simulink model "PMSM_SMO_ClosedLoop"  (R2026a)
settings: Solver=ode4  StopTime=.5  FixedStep=timing_h  MaxStep=1e-6
InitFcn:
  | pmsm_sensorless_v2_init(bdroot);
model workspace (MATLAB code in the model file + MAT data in the model file):
  T = 1e-6    (= 1e-06)
  MotorProfile = 'CHENSHA 200W / firmware profile revision 2'
  MotorSourceCommit = '48d6e86814ac6657b1313b4c92ef24c88f492e07'
  Pn = 200
  Un = 24
  Vdc = 24
  I_rated_rms = 11.5
  I_peak_rms = 23
  In = sqrt(2)*I_rated_rms
  I_peak = sqrt(2)*I_peak_rms
  n = 3000
  p = 5
  Rs = 0.105125
  Ld = 103.7615e-6    (= 0.0001037615)
  Lq = 103.7615e-6    (= 0.0001037615)
  Ls = Ld    (= 0.0001037615)
  phis = 0.06/(sqrt(2)*1.5*p)
  J = 32e-6    (= 3.2e-05)
  F = 0
  Kt = 1.5*p*phis
  Tn = 0.69
  T_peak = 1.38
  Iq_limit = 8
  accel_limit_rad_s2 = 1200
  speed_peak_rad_s = 335
  I_protection_A = 10
  Vbus_protection_high_V = 30
  Vbus_protection_low_V = 10
  RE = 10000
  rr = 2*pi/RE    (= 0.000628318530718)
  encoder_direction = -1
  fN = p*n/60    (= 250)
  wN = 2*pi*fN    (= 1570.79632679)
  ki_p = 0.8
  ki_i = 1
  fc = 20e3    (= 20000)
  Ts = 1/fc    (= 5e-05)
  dt = Ts    (= 5e-05)
  Ts_speed = 2*dt    (= 0.0001)
  w_sb = 2*pi*fN*1.2    (= 1884.95559215)
  fcb = 1000
  fwb = 50
  wc = 2*pi*fcb    (= 6283.18530718)
  wsc = 2*pi*fwb    (= 314.159265359)
  K = 30/pi    (= 9.54929658551)
  kp_w = 0.00069087230807625508    (= 0.000690872308076)
  ki_w = 0.04340878735241975    (= 0.0434087873524)
  ks_w = 0.98718608264211138    (= 0.987186082642)
  kp_id = 0.7539822368615503    (= 0.753982236862)
  ki_id = 879.64594300514204    (= 879.645943005)
  ks_id = 1.1309733552923253    (= 1.13097335529)
  kp_iq = 0.7539822368615503    (= 0.753982236862)
  ki_iq = 879.64594300514204    (= 879.645943005)
  ks_iq = 1.1309733552923253    (= 1.13097335529)
  Bm = 0
  uplimit_w = Kt*Iq_limit
  downlimit_w = -uplimit_w
  uplimit_id = Vdc/sqrt(3)
  downlimit_id = -uplimit_id
  uplimit_iq = Vdc/sqrt(3)
  downlimit_iq = -uplimit_iq
  teaching_Ts_speed = Ts_speed    (= 0.0001)
  teach_pwm_on = 0
  teach_pwm_cycles = 1
  decoupling_enabled = 1
  voltage_utilization = 0.96
  timing_on = 0
  timing_h = 1e-6    (= 1e-06)
  timing_control_sample = dt    (= 5e-05)
  timing_speed_sample = Ts_speed    (= 0.0001)
  timing_static_math = -1
  timing_carrier_y = [0 Ts/2 0]
  timing_adc_cfg = [0 0 0 1e-6 Ts 24.375e-6 1.1875e-6 1.5e-6 0 .5e-6 2]
  timing_pwm_cfg = [0 1e-6 Ts 24.375e-6 1.1875e-6 1.5e-6 0 5e-6 0 4000]
  dead_gate_on = 0
  dead_h = 1e-6    (= 1e-06)
  dead_gate_cfg = [0 1e-6 .5e-6]
  dead_comp_cfg = [0 .5e-6 Ts .05]
  dead_bridge_cfg = [p phis .01 0 .01 .7]
  sless_adc_mode = [1 0]
  sless_cfg = [0.105125 0.0001037615 5e-05 0.950604638176 0.469872645179 70 14 0.2 0.028048810878 0.777767679172 1332.66360365 888264.396098 2000 5 2 1.5 0.5 0.15]
  sless_closed_cfg = [5e-05 2.8875e-05 5 0.04 0.06 0.14 1200 6 6 0.18 0.02 0.04 0.02 0.08 0.000690872308076 0.0434087873524 0.987186082642 0.33941125497 0.0424264068712 2]
  sless_direction = 1
  sless_enabled = 1
  sless_v2_cfg = [6.25e-08 5e-05 0.0001 2.4375e-05 1.1875e-06 1.5e-06 0 0 3e-06 5e-06 2e-06 6e-05 7.5e-05 4.375e-07 0.012 0.6 0.05 0.05 5 2000 0.105125 0.0001037615 4500 2000 1.008 0.994 1.002 0.04 -0.02 0.005 20 12 0 0 0.25]
  sless_v2_interference_s = 0
  sless_voltage_cfg = [6.25e-08 5e-05 2.8875e-05 0.105125 0.0001037615 1]
undefined symbols (not defined in the file): DiscIntNeverNeededParam
libraries: simulink x3
(part 1 of 3)
Description:
  | CHENSHA 200W nominal motor profile from AxDr_L dev 48d6e86814ac6657b1313b4c92ef24c88f492e07. PI gains frozen from previous model. Current/PWM 20kHz, speed 10kHz. Bench iq command limit 8A. ABZ estimator, active protection and hardware sampling windows are not implemented.
settings Model: Creator=OptiPlex 7090  LastModifiedBy=lenovo
settings SimscapeCC: SimscapeLogDecimation=1  SimscapeNominalValues="[{\"value\":\"1\",\"unit\":\"A\"},{\"value\":\"1\",\"unit\":\"bar\"},{\"value\":\"1\",\"unit\":\"cm^2\"},{\"value\":\"1\",\"unit\":\"cm^3/s\"},{\"value\":\"1\",\"unit\":\"kJ/kg\"},{\"value\":\"1\",\"unit\":\"kW\"},{\"value\":\"1\",\"unit\":\"l\"},{\"value\":\"1\",\"unit\":\"N\"},{\"value\":\"1\",\"unit\":\"N*m\"},{\"value\":\"1\",\"unit\":\"V\"}]"  SimscapeLogDataHistory=5000  SimscapeLogType=none

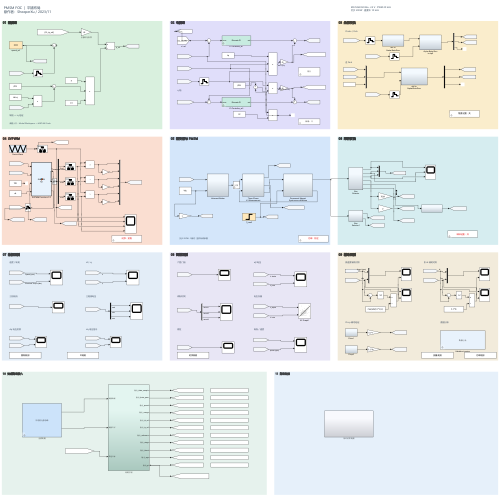
[thumbnail: Simulink's stored preview of the top-level diagram]
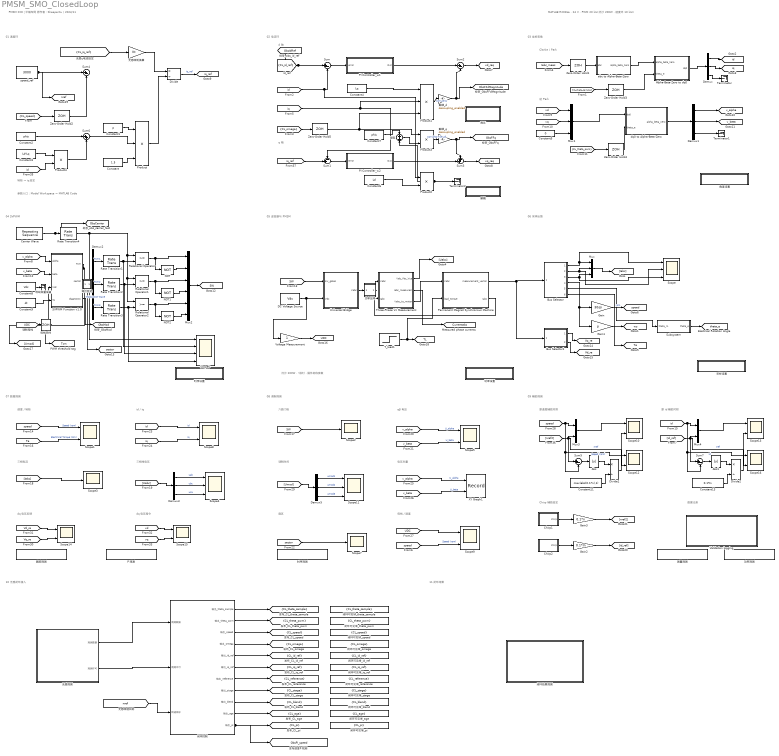
== system PMSM_SMO_ClosedLoop ==
  note: 参数入口：Model Workspace → MATLAB Code
  note: 07 数据观测
  note: 04 SVPWM
  note: 01 速度环
  note: 沉沙 200W · 5极对 · 固件标称参数
  note: 02 电流环
  note: 03 坐标变换
  note: 05 逆变器与 PMSM
  note: PMSM FOC  |  平铺布局
      | 原作者：SheeperXu / 2023/11
  note: 06 采样反馈
  note: MATLAB R2026a · 24 V · PWM 20 kHz
      | 沉沙 200W · 速度环 10 kHz
  note: 08 调制观测
  note: 09 辅助观测
  note: Clarke / Park
  note: 逆 Park
  note: d 轴
  note: q 轴
  note: 转矩 → iq 给定
  note: 速度 / 转矩
  note: id / iq
  note: 三相电流
  note: 三相线电压
  note: dq 电压反馈
  note: dq 电压指令
  note: 六路门极
  note: αβ 电压
  note: 调制时间
  note: 电压矢量
  note: 扇区
  note: 母线 / 速度
  note: 原速度辅助对照
  note: 原 id 辅助对照
  note: Chirp 辅助给定
  note: 数据记录
  note: 10 无感闭环接入
  note: 11 闭环结果
  Abs : Abs  SaturateOnIntegerOverflow=off
  Abs1 : Abs  SaturateOnIntegerOverflow=off
  Alpha-Beta-Zero to dq0 : Subsystem
  Bus Selector : Subsystem
  Bus Selector1 : Subsystem
  Carrier Wave : simulink/Sources/Repeating Sequence  rep_seq_t=[0 Ts/2 Ts]  rep_seq_y=timing_carrier_y
  Chirp1 : Subsystem
  Chirp2 : Subsystem
  Constant : Constant  Value=1.5
  Constant1 : Constant  Value=p
  Constant11 : Constant  Value=max(abs(0.1*n),1)
  Constant13 : Constant  Value=0.1*In
  Constant2 : Constant  Value=phis
  Constant3 : Constant  Value=Ld-Lq
  Constant4 : Constant  Value=Lq
  Constant5 : Constant  Value=0
  Constant6 : Constant  Value=Ld
  Constant7 : Constant  Value=phis
  Constant8 : Constant  Value=Vdc
  Constant9 : Constant  Value=dt
  DC Voltage Source : Constant  Value=Vdc
  Demux{,1..3,5} (5 alike) : Demux  Outputs=3
  Divide : Product  Inputs=*/
  Divide1 : Product  Inputs=*/
  Divide2 : Product  Inputs=*/
  Gain : Gain  Gain=30/pi
  Gain1 : Gain  Gain=p
  Gain2 : Gain  Gain=0.1*In
  Gain3 : Gain  Gain=0.1*n
  Mux : Mux  Inputs=3
  Mux1 : Mux  Inputs=3
  Mux2 : Mux  Inputs=6
  Mux3 : Mux  Inputs=2
  Mux4 : Mux  Inputs=2
  NOT : Logic  Operator=NOT  IconShape=distinctive  AllPortsSameDT=off  OutDataTypeStr=boolean
  NOT1 : Logic  Operator=NOT  IconShape=distinctive  AllPortsSameDT=off  OutDataTypeStr=boolean
  NOT2 : Logic  Operator=NOT  IconShape=distinctive  AllPortsSameDT=off  OutDataTypeStr=boolean
  PI Controller_w1 : Subsystem  mask{Kp=kp_id, Ki=ki_id, Ks=ks_id, uplimit=uplimit_id, downlimit=downlimit_id, SampleTime=timing_control_sample}
      mask prompts: uplimit "Up_Limit"; downlimit "Down_Limit"; SampleTime "Sample_Time(s)"
      mask DialogControl DescTextVar Prompt: PI Controller
      mask DialogControl ParameterGroupVar Prompt: 参数
      mask DialogControl Control2 Prompt: PI Controller Parameters
      mask Display:
      | disp('Discrete PI');
      | port_label('input',1,'error');
      | port_label('output',1,'out');
  PI Controller_w2 : Subsystem  mask{Kp=kp_iq, Ki=ki_iq, Ks=ks_iq, uplimit=uplimit_iq, downlimit=downlimit_iq, SampleTime=timing_control_sample}
      mask prompts: uplimit "Up_Limit"; downlimit "Down_Limit"; SampleTime "Sample_Time(s)"
      mask DialogControl DescTextVar Prompt: PI Controller
      mask DialogControl ParameterGroupVar Prompt: 参数
      mask DialogControl Control2 Prompt: PI Controller Parameters
      mask Display:
      | disp('Discrete PI');
      | port_label('input',1,'error');
      | port_label('output',1,'out');
  PI观测 : Subsystem  mask(PI观测){}
      mask help: 每组顺序：P / I / 限幅前 / 限幅后。速度环单位N*m；电流环单位V。
      settings: OpenFcn=open_system([gcb '/总览']);
      mask Display: disp('PI观测');
  Permanent Magnet Synchronous Machine : Subsystem
  Product : Product  Inputs=3  SampleTime=timing_static_math
  Product1 : Product  Inputs=3
  Product2 : Product
  Product3 : Product
  Product4 : Product
  Rate Transition{1..4} (4 alike) : RateTransition  Deterministic=off
  Relational Operator : RelationalOperator  OutDataTypeStr=boolean  RndMeth=Simplest  InputSameDT=off
  Relational Operator1 : RelationalOperator  OutDataTypeStr=boolean  RndMeth=Simplest  InputSameDT=off
  Relational Operator2 : RelationalOperator  OutDataTypeStr=boolean  RndMeth=Simplest  InputSameDT=off
  SVPWM Function v1.0 : MATLAB Function  TreatAsAtomicUnit=on
  Scope : Scope  NumInputPorts=3
      settings: ActiveDisplayYMinimum=-2.21804  ActiveDisplayYMaximum=2.01558
  Scope{1,5,8..10,12..16} (10 alike) : Scope  NumInputPorts=2
      Scope1 settings: ActiveDisplayYMinimum=-389.77916  ActiveDisplayYMaximum=3379.29942  DataLoggingVariableName=ScopeData3
      Scope10 settings: ActiveDisplayYMinimum=-396.87  ActiveDisplayYMaximum=406.58362  DataLoggingVariableName=ScopeData14
      Scope12 settings: ActiveDisplayYMinimum=-396.37475  ActiveDisplayYMaximum=405.982  DataLoggingVariableName=ScopeData15
      Scope13 settings: ActiveDisplayYMinimum=-1.103599846952628  ActiveDisplayYMaximum=7.8207274341227286  DataLoggingVariableName=ScopeData18
      Scope14 settings: ActiveDisplayYMinimum=-20.0031  ActiveDisplayYMaximum=19.99997  DataLoggingVariableName=ScopeData16
      Scope15 settings: ActiveDisplayYMinimum=-4.01522  ActiveDisplayYMaximum=14.86532  DataLoggingVariableName=ScopeData17
      Scope16 settings: ActiveDisplayYMinimum=-1.103599846952628  ActiveDisplayYMaximum=7.8207274341227286  DataLoggingVariableName=ScopeData19
      Scope5 settings: ActiveDisplayYMinimum=-10.001349433509255  ActiveDisplayYMaximum=9.60909342723076  DataLoggingVariableName=ScopeData7
      Scope8 settings: ActiveDisplayYMinimum=-0.61064  ActiveDisplayYMaximum=0.4372  DataLoggingVariableName=ScopeData10
      Scope9 settings: ActiveDisplayYMinimum=14  ActiveDisplayYMaximum=34  DataLoggingVariableName=ScopeData11
  Scope11 : Scope  NumInputPorts=3
      settings: ActiveDisplayYMinimum=2E-6  ActiveDisplayYMaximum=2.5E-5  DataLoggingVariableName=ScopeData13
  Scope2 : Scope
      settings: ActiveDisplayYMinimum=-0.125  ActiveDisplayYMaximum=1.125  DataLoggingVariableName=ScopeData4
  Scope3 : Scope
      settings: ActiveDisplayYMinimum=-14.55664  ActiveDisplayYMaximum=14.56696  DataLoggingVariableName=ScopeData5
  Scope4 : Scope  NumInputPorts=3
      settings: ActiveDisplayYMinimum=-30.00473  ActiveDisplayYMaximum=30.00442  DataLoggingVariableName=ScopeData6
  Scope6 : Scope  NumInputPorts=4
      settings: ActiveDisplayYMinimum=-3E-6  ActiveDisplayYMaximum=2.8E-5  DataLoggingVariableName=ScopeData8
  Scope7 : Scope
      settings: ActiveDisplayYMinimum=0.375  ActiveDisplayYMaximum=6.625  DataLoggingVariableName=ScopeData9
  Subsystem : Subsystem
  Sum{,2,4..5,7} (5 alike) : Sum  Inputs=|+-
  Sum1 : Sum  Inputs=-+|
  Sum3 : Sum  Inputs=++|
  Sum6 : Sum  Inputs=|++  SampleTime=timing_static_math
  T_load1 : Step  Time=.34  FinalValue=.207  SampleTime=timing_control_sample
  Terminator : Terminator
  Terminator1 : Terminator
  Terminator2 : Terminator
  Three-Phase V-I Measurement : Subsystem
  Universal Bridge : Subsystem
  Validation logging : Subsystem
      mask help: 原日志保留；obs_*为新增日志。默认dt的控制量记录不能用来判断PWM开关纹波。功率与门极的快速日志按T采样。
      mask Display: disp('数据记录');
  Voltage Measurement : Gain
  XY Graph1 : Record  NumPorts=2.0  FileSettingsInternal="{\"entries\":[{\"content\":{\"excelSettings\":{\"content\":{},\"type\":\"Streamout.ExcelSettings\"},\"parquetSettings\":{\"content\":{},\"type\":\"Streamout.ParquetSettings\"}},\"type\":\"Streamout.FileSettingStorage\",\"uuid\":\"\"}],\"packageUris\":[\"http:\\/\\/schema.mathworks.com\\/mf0\\/streamout_blocks\\/R2020a\"],\"version\":\"1.0\"}"  FrameSettings=[0, 0]  Layout=[1 1]  SignalsInternal="{\"entries\":[{\"content\":{\"signals\":[{\"content\":{\"blockPath\":[],\"dimensions\":[1],\"domain\":\"\",\"lineColor\":\"#a2142f\",\"plots\":[ 1 ],\"port\":1,\"sid\":[\"\"],\"signalID\":1,\"signalName\":\"U_alpha\"},\"type\":\"RecordBlkView.Signal\",\"uuid\":\"\"},{\"content\":{\"blockPath\":[],\"dimensions\":[1],\"domain\":\"\",\"lineColor\":\"#139fff\",\"plots\":[ 1 ],\"port\":2,\"sid\":[\"\"],\"signalID\":2,\"signalName\":\"U_beta\"},\"type\":\"RecordBlkView.Signal\",\"uuid\":\"\"}]},\"type\":\"RecordBlkView.InputSignals\",\"uuid\":\"\"}],\"packageUris\":[\"http:\\/\\/schema.mathworks.com\\/mf0\\/streamout_blocks\\/R2020a\"],\"version\":\"1.0\"}"  VisualizationBindings="{\"xyplotplugin\":{\"info\":[{\"series\":[{\"bindingParametersList\":[{\"parameter\":\"X-Axis\",\"signalID\":1,\"signalName\":\"U_alpha\"},{\"parameter\":\"Y-Axis\",\"signalID\":2,\"signalName\":\"U_beta\"}],\"seriesID\":0}],\"subplotID\":1}]}}"  CompatibilityTag=XY  st=-1
  Zero-Order Hold{1,3..5} (4 alike) : ZeroOrderHold  SampleTime=timing_control_sample
  Zero-Order Hold2 : ZeroOrderHold  SampleTime=timing_speed_sample
  abc to Alpha-Beta-Zero : Subsystem
  dq0 to Alpha-Beta-Zero : Subsystem
  speed_ref : Constant  Value=3000
  功率压降 : Subsystem
      mask help: 周期平均误差教学模型，非逐开关沿死区/二极管模型。正相电流定义为逆变器流向电机。每Ts保持电流，压降=开关死区项+导通电阻项，去除共模后从理想相电压扣除。0.5us来自AxDr_L dev配置；Ron、Vf和过零平滑均为演示参数。忽略最小脉宽、钳位、二极管瞬态和开关损耗。
      mask Display: disp('压降');
  功率观测 : Subsystem  mask(功率观测){}
      mask help: 相电压按T采样；平均压降按dt记录；功率统计请运行run_observation_demo。
      settings: OpenFcn=open_system([gcb '/总览']);
      mask Display: disp('功率观测');
  功率设置 : Subsystem  mask(功率设置){dead_on=off, dead_us=0.5, drop_on=on, ron=0.01, vf=0.69999999999999996, blend_A=0.1, pwm_period=Ts, gate_on=on, comp_on=off, gate_us=0.5, comp_us=0.5, hysteresis_A=0.05, zero_A=0.01}
      mask prompts: dead_on "死区平均压降"; dead_us "死区 [μs，固件目标]"; drop_on "器件导通压降"; ron "等效导通电阻 [Ω，演示]"; vf "续流压降 [V，演示，仅随死区项计入]"; blend_A "过零平滑电流 [A，演示]"; gate_on "门极死区（实际空白与续流）"; comp_on "死区补偿（测量电流极性）"; gate_us "门极死区 [μs，固件配置]"; comp_us "补偿死区 [μs，可作失配对照]"; hysteresis_A "补偿极性滞环 ±[A，演示]"; zero_A "续流近零数值带 ±[A，演示]"
      mask help: 门极死区：下降沿立即关断，上升沿延迟；三相浮置星点按实际门极及相电流方向续流。0.5us是定时器编程配置，不含未知驱动传播差异。近零带为数值近似，当前仅适用于Ld=Lq。补偿使用测量电流和测量角，按Vbus*tcomp/Ts加相电压修正，先合入dq再统一限压及回算。旧平均死区与门极死区互斥；详细模式的drop_on在桥内计算Ron/Vf，不再叠加旧平均压降。
      mask init:
      | validateattributes(dead_us,{'double'},{'scalar','real','finite','nonnegative','<',pwm_period*1e6/10});
      | validateattributes(ron,{'double'},{'scalar','real','finite','nonnegative'});
      | validateattributes(vf,{'double'},{'scalar','real','finite','nonnegative'});
      | validateattributes(blend_A,{'double'},{'scalar','real','finite','positive'});
      mask Display: if gate_on&&comp_on, color('red');disp('功率：补偿');elseif gate_on, color('red');disp('功率：死区');elseif dead_on||drop_on,disp('功率：平均');else,disp('功率：理想');end
  无感观测 : Subsystem  mask(Local sensorless nonideal v2){enabled=on, R_hat=0.105125, L_hat=0.00010376150000000001, Kslide_V=14, boundary_A=0.20000000000000001, emf_filter_hz=800, pll_fn_hz=150, pll_zeta=0.70699999999999996, omega_limit_rad_s=2000, direction=1, derived_a=0.95060463817554253, derived_b=0.46987264517914396, derived_kp=1332.6636036527902, derived_ki=888264.39609804214, analog_hat_hz=4500, digital_hat_hz=2000, deadtime_hat_us=.4375, ron_hat_ohm=.012, vf_hat_V=.6, observer_budget_us=3, foc_budget_us=5, guard_us=2, gain_hat_ABC=[1.008 .994 1.002], bias_hat_ABC_A=[.04 -.02 .005], adc_span_A=20, adc_bits=12, packet_phase_limit_deg=5}
      mask prompts: enabled "旁路观测"; R_hat "观测相电阻 [Ω]"; L_hat "观测电感 [H]"; Kslide_V "滑模注入 [V]"; boundary_A "边界层 [A]"; emf_filter_hz "反电动势滤波 [Hz]"; pll_fn_hz "PLL自然频率 [Hz]"; pll_zeta "PLL阻尼比"; omega_limit_rad_s "电角速度限值 [rad/s]"; direction "旋转方向 ±1 / 0"; derived_a "离散 a"; derived_b "离散 b [A/V]"; derived_kp "PLL Kp [1/s]"; derived_ki "PLL Ki [1/s²]"; analog_hat_hz "估计模拟低通 [Hz]"; digital_hat_hz "数字低通 [Hz]"; deadtime_hat_us "估计死区 [μs]"; ron_hat_ohm "估计导通电阻 [Ω]"; vf_hat_V "估计二极管压降 [V]"; observer_budget_us "观测计算预算 [μs]"; foc_budget_us "FOC计算预算 [μs]"; guard_us "截止期裕量 [μs]"; gain_hat_ABC "观测标定增益 ABC"; bias_hat_ABC_A "观测标定零偏 ABC [A]"; adc_span_A "已配置ADC正负量程 [A]"; adc_bits "已配置ADC位数"; packet_phase_limit_deg "发布瞬时相位门槛 [电角度°]"
      mask Display: disp('非理想无感旁路')
  无感转矩换算 : Gain  Gain=Kt
  时序观测 : Subsystem  mask(时序观测){}
      mask help: 门极按求解步长T记录；当前死区仅平均压降，不产生门极空白。
      settings: OpenFcn=open_system([gcb '/总览']);
      mask Display: disp('时序观测');
  时序设置 : Subsystem  Tag=TeachingControl  mask(时序设置){speed_on=off, speed_divider=20, pwm_on=off, pwm_cycles=1, real_on=on, window_on=off, invalid_hold_on=off, trigger_us=24.375, sync_us=0, compute_us=8, settle_us=0.5, update_mode=峰谷双更新（RCR=0）, grid_divider=1}
      mask prompts: speed_on "速度分频"; speed_divider "速度周期 / 电流周期"; pwm_on "输出延迟"; pwm_cycles "延迟周期数 [× dt]"; real_on "真实时序（顺序采样与CCR生效）"; window_on "低侧采样窗口（无效样本置零演示）"; invalid_hold_on "无效时保持上次有效值（策略对照）"; trigger_us "触发相位 [μs，24.375为待实测假设]"; sync_us "触发附加等待 [μs，演示]"; compute_us "JEOS至CCR写入 [μs，演示]"; settle_us "低侧导通稳定等待 [μs，演示]"; update_mode "CCR预装载生效边界"
      mask help: 真实时序：C/B/A顺序采样，JEOS执行原控制器，计算后写CCR，下一UEV生效。RCR=0按峰谷双更新；24.375us触发相位是源码推导假设，CC4路由及下降沿须实测。计算5us、稳定等待0.5us均为演示值。窗口检查整个采样孔径；无效样本置零仅为低侧不可观测演示，保持策略不是当前固件行为。真实模式使用62.5ns网格，仍无门极死区/二极管模型。与旧整周期延迟互斥。
      mask TypeOptions update_mode: 峰谷双更新（RCR=0） | 仅谷底（对照）
      mask Display: if real_on, color('red'); disp('时序：实物'); elseif speed_on||pwm_on, disp('时序：教学'); else, disp('时序：理想'); end
  母线常量保留 : Terminator
  母线采样 : ZeroOrderHold  SampleTime=timing_control_sample
  测量观测 : Subsystem  mask(测量观测){}
      mask help: 真实电流、测量电流及误差分别显示。误差为measured - true；包含滤波相位滞后。
      settings: OpenFcn=open_system([gcb '/总览']);
      mask Display: disp('测量观测');
  磁链 : Sum
  角度设置 : Subsystem  Tag=TeachingControl  mask(角度设置){bias_on=off, bias_deg=2, quant_on=off, step_deg=0.18, delay_on=off, delay_cycles=1}
      mask prompts: bias_on "角度偏置"; bias_deg "偏置 [电角度 °]"; quant_on "角度量化"; step_deg "量化步长 [电角度 °]"; delay_on "角度延迟"; delay_cycles "延迟周期数 [× dt]"
      mask help: 运行前设置。使用电角单位；偏置与量化为电角度，延迟按 dt 整周期。全部关闭时直通原角度；暂不实现角度预测、传感器接口或丢帧。
      mask init:
      | validateattributes(bias_deg,{'double'},{'scalar','real','finite'});
      | validateattributes(step_deg,{'double'},{'scalar','real','finite','positive','<=',360});
      | validateattributes(delay_cycles,{'double'},{'scalar','real','finite','integer','>=',1,'<=',20});
      mask Display: if bias_on||quant_on||delay_on, color('red'); disp('角度设置：开'); else, color('black'); disp('角度设置：关'); end
  解耦 : Subsystem  mask{enabled=on}
      mask prompts: enabled "dq解耦与反电动势前馈（运行前选择）"
      mask help: 开：vd_ff=-we*Lq*iq；vq_ff=we*(phis+Ld*id)。关：两个前馈均为零。最终限压与抗饱和始终启用。
      mask Display: if enabled, disp('解耦：开'); else, disp('解耦：关'); end
  解耦_d : Gain  Gain=decoupling_enabled
  解耦_q : Gain  Gain=decoupling_enabled
  跟踪观测 : Subsystem  mask(跟踪观测){}
      mask help: 按单位分轴；主控制给定，无Chirp辅助参考。
      settings: OpenFcn=open_system([gcb '/总览']);
      mask Display: disp('跟踪观测');
  输出延迟 : Subsystem  mask{real_mode=strcmp(get_param([bdroot '/时序设置'],'real_on'),'on')}
      mask help: 理想/旧整周期延迟或真实CCR预装载分支。真实时序在时序设置中启用，包含CCR量化、计算完成与更新边界。
      mask Display: disp('更新');
  采样设置 : Subsystem  Tag=TeachingControl  mask(采样设置){bias_on=on, bias_A=[0.050000000000000003;-0.029999999999999999;0], gain_on=on, phase_gain=[1.01;0.98999999999999999;1], noise_on=on, noise_rms=0.02, noise_seed=20261016, adc_on=on, adc_bits=12, adc_span=20, filter_on=on, filter_hz=2000, delay_on=off, delay_cycles=1, control_period=dt, analog_on=on, analog_hz=5000, numerical_step=T, real_mode=strcmp(get_param([bdroot '/时序设置'],'real_on'),'on')}
      mask prompts: bias_on "零偏"; bias_A "三相零偏 [A]"; gain_on "增益误差"; phase_gain "三相增益"; noise_on "采样噪声"; noise_rms "每相噪声 RMS [A]"; noise_seed "随机种子"; adc_on "ADC 量化与饱和"; adc_bits "分辨率 [bit，演示]"; adc_span "双极量程 ± [A]"; filter_on "数字低通"; filter_hz "等效低通频率 [Hz]"; delay_on "采样传递延迟"; delay_cycles "延迟周期数 [× dt]"; analog_on "模拟低通（采样前）"; analog_hz "模拟一阶截止频率 [Hz，演示]"
      mask help: 运行前设置；参数均为演示值。等效电流域模型：增益/零偏/采样噪声 → 同步采样 → 量化/饱和 → 数字滤波 → 整周期传递延迟。未模拟分流电阻、模拟 RC、放大器或有效采样窗口。全部关闭时直通原信号。 新增模拟一阶低通在同步采样之前，初始状态为0；模拟/数字滤波独立开关。RC与放大器实际参数待原理图确认。
      mask init:
      | validateattributes(bias_A,{'double'},{'vector','numel',3,'real','finite'});
      | validateattributes(phase_gain,{'double'},{'vector','numel',3,'real','finite','positive'});
      | validateattributes(noise_rms,{'double'},{'scalar','real','finite','nonnegative'});
      | validateattributes(noise_seed,{'double'},{'scalar','real','finite','integer','>=',1,'<=',4294967293});
      | validateattributes(adc_bits,{'double'},{'scalar','real','finite','integer','>=',1,'<=',24});
      | validateattributes(adc_span,{'double'},{'scalar','real','finite','positive'});
      | validateattributes(filter_hz,{'double'},{'scalar','real','finite','positive','<',1/(2*control_period)});
      | validateattributes(delay_cycles,{'double'},{'scalar','real','finite','integer','>=',1,'<=',20});
      | validateattributes(analog_hz,{'double'},{'scalar','real','finite','positive'});
      | assert(2*pi*analog_hz*numerical_step<1,'Analog filter requires a smaller numerical step T.');
      mask DialogControl error Prompt: 误差
      mask DialogControl adc Prompt: ADC
      mask DialogControl filter Prompt: 滤波与延迟
      mask Display: if bias_on||gain_on||noise_on||adc_on||filter_on||delay_on||analog_on, color('red'); disp('采样设置：开'); else, color('black'); disp('采样设置：关'); end
  闭环可见域_age : GotoTagVisibility  GotoTag=CL_age
  闭环可见域_blend : GotoTagVisibility  GotoTag=CL_blend
  闭环可见域_id_ref : GotoTagVisibility  GotoTag=CL_id_ref
  闭环可见域_iq_ref : GotoTagVisibility  GotoTag=CL_iq_ref
  闭环可见域_omega : GotoTagVisibility  GotoTag=CL_omega
  闭环可见域_pi : GotoTagVisibility  GotoTag=CL_pi
  闭环可见域_reference : GotoTagVisibility  GotoTag=CL_reference
  闭环可见域_speed : GotoTagVisibility  GotoTag=CL_speed
  闭环可见域_stage : GotoTagVisibility  GotoTag=CL_stage
  闭环可见域_theta_pwm : GotoTagVisibility  GotoTag=CL_theta_pwm
  闭环可见域_theta_sample : GotoTagVisibility  GotoTag=CL_theta_sample
  闭环控制 : Subsystem
  闭环结果观测 : Subsystem
  限压 : Subsystem
      mask help: 输入：PI轴限幅输出+前馈；方向保持的dq圆限幅，Vmax=0.96*max(Vbus,0)/sqrt(3)。输出vd/vq；最终残差Vfinal-Vrequest回到PI，和原轴限幅残差合并，仅回算一次。
      mask Display: disp('限压');
  tag scope: CL_age=scoped, CL_blend=scoped, CL_id_ref=scoped, CL_iq_ref=scoped, CL_omega=scoped, CL_pi=scoped, CL_reference=scoped, CL_speed=scoped, CL_stage=scoped, CL_theta_pwm=scoped, CL_theta_sample=scoped, Currentabc=global, ObsCarrier=global, ObsFFdMagnitude=global, ObsFFq=global, ObsIdRef=global, ObsMod=global, ObsPI_speed=global, SW=global, TL=global, Tcm=global, Te=global, UDC=global, Vd_re=global, Vq_re=global, id=global, iq=global, iq_ref=global, nref=global, sector=global, speed=global, theta_e=global, v_alpha=global, v_beta=global, vd_req=global, vq_req=global, ws=global
  wires:
  Sum5/1 -> Abs/1
  Sum7/1 -> Abs1/1
  abc to Alpha-Beta-Zero/1(alpha_beta_zero) -> Alpha-Beta-Zero to dq0/1(alpha_beta_zero)
  Zero-Order Hold3/1 -> Alpha-Beta-Zero to dq0/2(theta_e)
  Permanent Magnet Synchronous Machine/1(measurement_vector) -> Bus Selector/1(measurement_vector), Bus Selector1/1(measurement_vector)
  Alpha-Beta-Zero to dq0/1(dq0) -> Demux/1
  dq0 to Alpha-Beta-Zero/1(alpha_beta_zero) -> Demux1/1
  SVPWM Function v1.0/1(Tcm) -> [Umod], [Tcm], 输出延迟/1(指令)  "Modulation Wave"
  [Uabc] -> Demux3/1
  [Umod] -> Demux5/1
  Product/1 -> Divide/2
  Abs/1 -> Divide1/1
  Constant11/1 -> Divide1/2
  Abs1/1 -> Divide2/1
  Constant13/1 -> Divide2/2
  Subsystem/1(theta_e) -> [theta_e]
  Bus Selector/4(signal_4) -> Gain/1, Gain1/1
  Chirp2/1(chirp) -> Gain2/1
  Chirp1/1(chirp) -> Gain3/1
  Mux/1 -> [Iabc]
  Gain1/1 -> [ws]
  Demux1/1 -> [v_alpha]
  Demux1/2 -> [v_beta]
  Mux2/1 -> [SW]
  SVPWM Function v1.0/2(sector) -> [sector]
  Bus Selector1/1(signal_7) -> [Vq_re]
  Bus Selector1/2(signal_8) -> [Vd_re]
  Voltage Measurement/1 -> [UDC]
  T_load1/1 -> [TL], Permanent Magnet Synchronous Machine/2(load_torque)
  Demux/1 -> [id]
  Gain2/1 -> [id_ref]
  Gain3/1 -> [nref2]
  Demux/2 -> [iq]
  Three-Phase V-I Measurement/1(Vab_Vbc_Vca) -> [Uabc]
  Bus Selector/6(signal_6) -> [Te]
  Gain/1 -> [speed]  "rpm"
  Sum2/1 -> [vd_req]
  Sum3/1 -> [vq_req]
  Divide/1 -> [iq_ref]  "iq_ref"
  Bus Selector/1(signal_1) -> Mux/1, Scope/1
  Bus Selector/2(signal_2) -> Mux/2, Scope/2
  Bus Selector/3(signal_3) -> Mux/3, Scope/3
  [vd] -> Mux1/1
  [vq] -> Mux1/2
  Constant5/1 -> Mux1/3
  Relational Operator/1 -> Mux2/1, NOT/1
  NOT/1 -> Mux2/2
  Relational Operator1/1 -> Mux2/3, NOT1/1
  NOT1/1 -> Mux2/4
  Relational Operator2/1 -> Mux2/5, NOT2/1
  NOT2/1 -> Mux2/6
  [speed] -> Scope12/1, Sum5/2, Mux3/1  "Speed (rpm)"
  [nref2] -> Mux3/2, Scope12/2, Sum5/1  "nref"
  [id] -> Scope16/1, Sum7/2, Mux4/1  "id"
  [id_ref] -> Mux4/2, Scope16/2, Sum7/1  "iref"
  Sum/1 -> PI Controller_w1/1(error)
  Sum1/1 -> PI Controller_w2/1(error)
  Constant1/1 -> Product/1
  Sum6/1 -> Product/2
  Constant/1 -> Product/3
  Constant4/1 -> Product1/1
  [iq] -> Product1/2, Sum1/1
  Zero-Order Hold5/1 -> Product1/3, Product3/1
  [id] -> Product2/1, Sum/2
  Constant6/1 -> Product2/2
  Constant7/1 -> 磁链/1
  Constant3/1 -> Product4/1
  [id] -> Product4/2
  Demux2/1 -> Rate Transition1/1  "Tcm1"
  Demux2/2 -> Rate Transition2/1  "Tcm2"
  Demux2/3 -> Rate Transition3/1  "Tcm3"
  Carrier Wave/1 -> Rate Transition4/1, [ObsCarrier]
  Rate Transition4/1 -> Relational Operator1/1, Relational Operator2/1, Relational Operator/1, Scope6/1
  Rate Transition1/1 -> Relational Operator/2, Scope6/2
  Rate Transition2/1 -> Relational Operator1/2, Scope6/3
  Rate Transition3/1 -> Relational Operator2/2, Scope6/4
  [v_alpha] -> SVPWM Function v1.0/1(alpha)
  [v_beta] -> SVPWM Function v1.0/2(beta)
  Constant9/1 -> SVPWM Function v1.0/4(Ts)
  [speed] -> Scope1/1  "Speed (rpm)"
  [Te] -> Scope1/2  "Electrical Torque (Nm)"
  Mux3/1 -> Scope10/1
  Divide1/1 -> Scope10/2
  Demux5/1 -> Scope11/1  "umod1"
  Demux5/2 -> Scope11/2  "umod2"
  Demux5/3 -> Scope11/3  "umod3"
  Mux4/1 -> Scope13/1
  Divide2/1 -> Scope13/2
  [Vd_re] -> Scope14/1
  [Vq_re] -> Scope14/2
  [vd] -> Scope15/1
  [vq] -> Scope15/2
  [SW] -> Scope2/1
  [Iabc] -> Scope3/1
  Demux3/1 -> Scope4/1  "uab"
  Demux3/2 -> Scope4/2  "ubc"
  Demux3/3 -> Scope4/3  "uca"
  [v_alpha] -> Scope5/1  "U_alpha"
  [v_beta] -> Scope5/2  "U_beta"
  [sector] -> Scope7/1
  [id] -> Scope8/1  "id"
  [iq] -> Scope8/2  "iq"
  [UDC] -> Scope9/1
  [speed] -> Scope9/2  "Speed (rpm)"
  Bus Selector/5(signal_5) -> Subsystem/1(theta_m)
  [iq_ref] -> Sum1/2
  PI Controller_w1/1(Out) -> Sum2/1
  Product1/1 -> 解耦_d/1  "ws*Lq*iq"
  Product3/1 -> 解耦_q/1  "ws*(phis+id*Ld)"
  PI Controller_w2/1(Out) -> Sum3/2
  Zero-Order Hold2/1 -> Sum4/2
  Constant2/1 -> Sum6/1
  Product4/1 -> Sum6/2
  Demux/3 -> Terminator/1
  Demux1/3 -> Terminator1/1
  Product2/1 -> Terminator2/1, 磁链/2
  [SW] -> Universal Bridge/1(six_gates)
  [v_alpha] -> XY Graph1/1  "U_alpha"
  [v_beta] -> XY Graph1/2  "U_beta"
  [Iabc_meas] -> Zero-Order Hold1/1
  [CL_speed] -> Zero-Order Hold2/1
  [CL_theta_sample] -> Zero-Order Hold3/1
  [CL_theta_pwm] -> Zero-Order Hold4/1
  [CL_omega] -> Zero-Order Hold5/1
  Zero-Order Hold1/1 -> abc to Alpha-Beta-Zero/1(abc)
  Mux1/1 -> dq0 to Alpha-Beta-Zero/1(dq0)
  Zero-Order Hold4/1 -> dq0 to Alpha-Beta-Zero/2(theta_e)
  DC Voltage Source/1 -> Universal Bridge/2(Vdc), Voltage Measurement/1
  Three-Phase V-I Measurement/3(Vabc_to_motor) -> Permanent Magnet Synchronous Machine/1(Vabc)
  Permanent Magnet Synchronous Machine/2(Iabc) -> Three-Phase V-I Measurement/2(Iabc)
  Three-Phase V-I Measurement/2(Iabc_measured) -> [Currentabc]
  输出延迟/1(生效) -> Demux2/1
  Universal Bridge/1(Vabc) -> 功率压降/1(理想)
  功率压降/1(实际) -> Three-Phase V-I Measurement/1(Vabc)
  磁链/1 -> Product3/2
  解耦_d/1 -> Sum2/2, [ObsFFdMagnitude]
  解耦_q/1 -> Sum3/1, [ObsFFq]
  [UDC] -> 母线采样/1
  母线采样/1 -> SVPWM Function v1.0/3(Vdc)
  Constant8/1 -> 母线常量保留/1
  SVPWM Function v1.0/3(diagnostic) -> [ObsMod]
  [CL_id_ref] -> Sum/1, [ObsIdRef]
  无感观测/1(观测数据) -> 闭环控制/1(观测数据)
  无感观测/2(观测许可) -> 闭环控制/2(观测许可)
  闭环控制/1(输出_theta_sample) -> [CL_theta_sample]
  闭环控制/2(输出_theta_pwm) -> [CL_theta_pwm]
  闭环控制/3(输出_speed) -> [CL_speed]
  闭环控制/4(输出_omega) -> [CL_omega]
  闭环控制/5(输出_id_ref) -> [CL_id_ref]
  闭环控制/6(输出_iq_ref) -> [CL_iq_ref]
  闭环控制/7(输出_reference) -> [CL_reference]
  闭环控制/8(输出_stage) -> [CL_stage]
  闭环控制/9(输出_blend) -> [CL_blend]
  闭环控制/10(输出_age) -> [CL_age]
  [CL_iq_ref] -> 无感转矩换算/1
  无感转矩换算/1 -> Divide/1
  [nref] -> 闭环控制/3(转速目标)
  speed_ref/1 -> [nref], Sum4/1
  闭环控制/11(输出_pi) -> [ObsPI_speed], [CL_pi]

== system PMSM_SMO_ClosedLoop/Alpha-Beta-Zero to dq0 ==
  alpha_beta_zero : Inport
  theta_e : Inport  Port=2
  axis_0 : Fcn  Expr=u(3)
  axis_1 : Fcn  Expr=u(1)*cos(u(4))+u(2)*sin(u(4))
  axis_2 : Fcn  Expr=-u(1)*sin(u(4))+u(2)*cos(u(4))
  input_vector : Mux  Inputs=2
  result : Mux  Inputs=3
  dq0 : Outport
  wires:
  alpha_beta_zero/1 -> input_vector/1
  theta_e/1 -> input_vector/2
  input_vector/1 -> axis_1/1, axis_2/1, axis_0/1
  axis_1/1 -> result/1
  axis_2/1 -> result/2
  axis_0/1 -> result/3
  result/1 -> dq0/1

== system PMSM_SMO_ClosedLoop/Bus Selector ==
  measurement_vector : Inport
  signals : Demux  Outputs=8
  unused_7 : Terminator
  unused_8 : Terminator
  signal_1 : Outport
  signal_2 : Outport  Port=2
  signal_3 : Outport  Port=3
  signal_4 : Outport  Port=4
  signal_5 : Outport  Port=5
  signal_6 : Outport  Port=6
  wires:
  measurement_vector/1 -> signals/1
  signals/1 -> signal_1/1
  signals/2 -> signal_2/1
  signals/3 -> signal_3/1
  signals/4 -> signal_4/1
  signals/5 -> signal_5/1
  signals/6 -> signal_6/1
  signals/7 -> unused_7/1
  signals/8 -> unused_8/1

== system PMSM_SMO_ClosedLoop/Bus Selector1 ==
  measurement_vector : Inport
  signals : Demux  Outputs=8
  unused_{1..6} (6 alike) : Terminator
  signal_7 : Outport
  signal_8 : Outport  Port=2
  wires:
  measurement_vector/1 -> signals/1
  signals/7 -> signal_7/1
  signals/8 -> signal_8/1
  signals/1 -> unused_1/1
  signals/2 -> unused_2/1
  signals/3 -> unused_3/1
  signals/4 -> unused_4/1
  signals/5 -> unused_5/1
  signals/6 -> unused_6/1

== system PMSM_SMO_ClosedLoop/Chirp1 ==
  linear_chirp : Fcn  Expr=cos(pi*500/10*u(1)^2)
  sample : ZeroOrderHold  SampleTime=timing_control_sample
  sweep_time : simulink/Sources/Repeating Sequence  rep_seq_t=[0 10]  rep_seq_y=[0 10]
  chirp : Outport
  wires:
  sweep_time/1 -> linear_chirp/1
  linear_chirp/1 -> sample/1
  sample/1 -> chirp/1

== system PMSM_SMO_ClosedLoop/Chirp2 ==
  linear_chirp : Fcn  Expr=cos(pi*5000/10*u(1)^2)
  sample : ZeroOrderHold  SampleTime=timing_control_sample
  sweep_time : simulink/Sources/Repeating Sequence  rep_seq_t=[0 10]  rep_seq_y=[0 10]
  chirp : Outport
  wires:
  sweep_time/1 -> linear_chirp/1
  linear_chirp/1 -> sample/1
  sample/1 -> chirp/1

== system PMSM_SMO_ClosedLoop/PI Controller_w1 ==
  error : Inport
  Add : Sum
  Discrete-Time Integrator : DiscreteIntegrator  IntegratorMethod=Integration: Backward Euler  SampleTime=timing_control_sample  LimitOutput=on  UpperSaturationLimit=uplimit  LowerSaturationLimit=downlimit  ICPrevOutput=DiscIntNeverNeededParam  ICPrevScaledInput=DiscIntNeverNeededParam
  Gain : Gain  Gain=Ks
  Ki : Gain  Gain=Ki
  Kp : Gain  Gain=Kp
  Saturation : Saturate  UpperLimit=uplimit  LowerLimit=downlimit
  Scope2 : Scope
      settings: ActiveDisplayYMinimum=-0.32149  ActiveDisplayYMaximum=0.29616
  Scope3 : Scope
      settings: ActiveDisplayYMinimum=-0.21306  ActiveDisplayYMaximum=0.20509  DataLoggingVariableName=ScopeData2
  Sum : Sum  Inputs=+|--
  Sum1 : Sum  Inputs=|+-
  Zero-Order Hold : ZeroOrderHold  SampleTime=timing_control_sample
  回算修正 : Gain  Gain=-1
  回算观测 : Mux  Inputs=2
  观测汇总 : Mux
  记录_obs_aw_d : ToWorkspace  VariableName=obs_aw_d  SaveFormat=Timeseries  SampleTime=timing_control_sample
  记录_obs_pi_d : ToWorkspace  VariableName=obs_pi_d  SaveFormat=Timeseries  SampleTime=timing_control_sample
  Out : Outport
  tag scope: ObsCorrection_d=global, ObsPI_d=global
  wires:
  Discrete-Time Integrator/1 -> Add/2, Scope3/1, 观测汇总/2
  Ki/1 -> Discrete-Time Integrator/1
  Sum1/1 -> Ki/1
  Gain/1 -> Sum1/2, 回算修正/1
  Sum/1 -> Gain/1
  Saturation/1 -> Out/1, Sum/2, 观测汇总/4
  Add/1 -> Saturation/1, Sum/1, 观测汇总/3
  Zero-Order Hold/1 -> Scope2/1, Add/1, 观测汇总/1
  error/1 -> Kp/1, Sum1/1
  Kp/1 -> Zero-Order Hold/1
  观测汇总/1 -> [ObsPI_d], 记录_obs_pi_d/1
  [ObsResidual_d] -> Sum/3, 回算观测/1
  回算修正/1 -> 回算观测/2, [ObsCorrection_d]
  回算观测/1 -> 记录_obs_aw_d/1

== system PMSM_SMO_ClosedLoop/PI Controller_w2 ==
  error : Inport
  Add : Sum
  Discrete-Time Integrator : DiscreteIntegrator  IntegratorMethod=Integration: Backward Euler  SampleTime=timing_control_sample  LimitOutput=on  UpperSaturationLimit=uplimit  LowerSaturationLimit=downlimit  ICPrevOutput=DiscIntNeverNeededParam  ICPrevScaledInput=DiscIntNeverNeededParam
  Gain : Gain  Gain=Ks
  Ki : Gain  Gain=Ki
  Kp : Gain  Gain=Kp
  Saturation : Saturate  UpperLimit=uplimit  LowerLimit=downlimit
  Scope2 : Scope
      settings: ActiveDisplayYMinimum=-0.81806  ActiveDisplayYMaximum=0.86163
  Scope3 : Scope
      settings: ActiveDisplayYMinimum=-2.70519  ActiveDisplayYMaximum=4.05153  DataLoggingVariableName=ScopeData2
  Sum : Sum  Inputs=+|--
  Sum1 : Sum  Inputs=|+-
  Zero-Order Hold : ZeroOrderHold  SampleTime=timing_control_sample
  回算修正 : Gain  Gain=-1
  回算观测 : Mux  Inputs=2
  观测汇总 : Mux
  记录_obs_aw_q : ToWorkspace  VariableName=obs_aw_q  SaveFormat=Timeseries  SampleTime=timing_control_sample
  记录_obs_pi_q : ToWorkspace  VariableName=obs_pi_q  SaveFormat=Timeseries  SampleTime=timing_control_sample
  Out : Outport
  tag scope: ObsCorrection_q=global, ObsPI_q=global
  wires:
  Kp/1 -> Zero-Order Hold/1
  error/1 -> Sum1/1, Kp/1
  Zero-Order Hold/1 -> Add/1, Scope2/1, 观测汇总/1
  Add/1 -> Sum/1, Saturation/1, 观测汇总/3
  Saturation/1 -> Sum/2, Out/1, 观测汇总/4
  Sum/1 -> Gain/1
  Gain/1 -> Sum1/2, 回算修正/1
  Sum1/1 -> Ki/1
  Ki/1 -> Discrete-Time Integrator/1
  Discrete-Time Integrator/1 -> Scope3/1, Add/2, 观测汇总/2
  观测汇总/1 -> [ObsPI_q], 记录_obs_pi_q/1
  [ObsResidual_q] -> Sum/3, 回算观测/1
  回算修正/1 -> 回算观测/2, [ObsCorrection_q]
  回算观测/1 -> 记录_obs_aw_q/1

== system PMSM_SMO_ClosedLoop/PI观测 ==
  note: 01 速度PI [N*m]
  note: 02 d轴PI [V]
  note: 03 q轴PI [V]
  dq请求与输出 [V] : Mux
  d轴PI : Scope
      settings: SampleTime=dt  Title=d轴PI [V]
  q轴PI : Scope
      settings: SampleTime=dt  Title=q轴PI [V]
  利用率 : Mux  Inputs=1
  前馈 [V] : Mux  Inputs=2
  可用电压 [V] : Mux  Inputs=1
  回算修正 [A] : Mux  Inputs=2
  总览 : Scope  NumInputPorts=10
      settings: SampleTime=dt  TimeSpan=0.12  ActiveDisplayString=10  Title=回算修正 [A]
  最终残差 [V] : Mux  Inputs=2
  速度PI : Scope
      settings: SampleTime=dt  Title=速度PI [N*m]
  饱和标志 : Mux  Inputs=1
  wires:
  [ObsPI_speed] -> 速度PI/1, 总览/1
  [ObsPI_d] -> d轴PI/1, 总览/2
  [ObsPI_q] -> q轴PI/1, 总览/3
  [ObsFFd] -> 前馈 [V]/1
  [ObsFFq] -> 前馈 [V]/2
  前馈 [V]/1 -> 总览/4
  [vd_req] -> dq请求与输出 [V]/1
  [vq_req] -> dq请求与输出 [V]/2
  [vd] -> dq请求与输出 [V]/3
  [vq] -> dq请求与输出 [V]/4
  dq请求与输出 [V]/1 -> 总览/5
  [ObsVmax] -> 可用电压 [V]/1
  可用电压 [V]/1 -> 总览/6
  [ObsUtilization] -> 利用率/1
  利用率/1 -> 总览/7
  [ObsSaturation] -> 饱和标志/1
  饱和标志/1 -> 总览/8
  [ObsResidual_d] -> 最终残差 [V]/1
  [ObsResidual_q] -> 最终残差 [V]/2
  最终残差 [V]/1 -> 总览/9
  [ObsCorrection_d] -> 回算修正 [A]/1
  [ObsCorrection_q] -> 回算修正 [A]/2
  回算修正 [A]/1 -> 总览/10

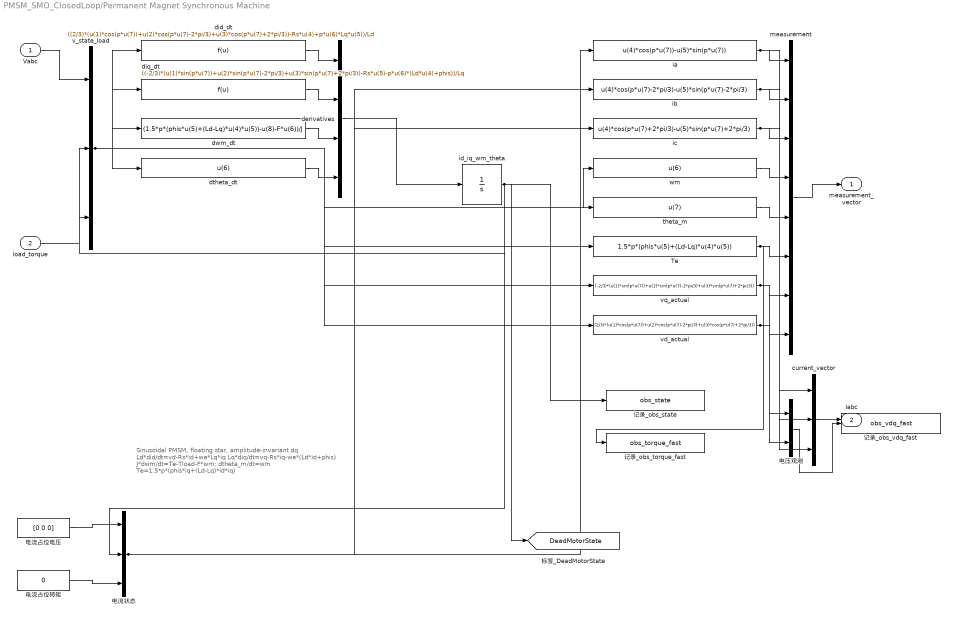
== system PMSM_SMO_ClosedLoop/Permanent Magnet Synchronous Machine ==
  note: Sinusoidal PMSM, floating star, amplitude-invariant dq.
      | Ld*did/dt=vd-Rs*id+we*Lq*iq
      | Lq*diq/dt=vq-Rs*iq-we*(Ld*id+phis)
      | J*dwm/dt=Te-Tload-F*wm; dtheta_m/dt=wm
      | Te=1.5*p*(phis*iq+(Ld-Lq)*id*iq)
  Vabc : Inport
  load_torque : Inport  Port=2
  Te : Fcn  Expr=1.5*p*(phis*u(5)+(Ld-Lq)*u(4)*u(5))
  current_vector : Mux  Inputs=3
  derivatives : Mux
  did_dt : Fcn  Expr=((2/3)*(u(1)*cos(p*u(7))+u(2)*cos(p*u(7)-2*pi/3)+u(3)*cos(p*u(7)+2*pi/3))-Rs*u(4)+p*u(6)*Lq*u(5))/Ld
  diq_dt : Fcn  Expr=((-2/3)*(u(1)*sin(p*u(7))+u(2)*sin(p*u(7)-2*pi/3)+u(3)*sin(p*u(7)+2*pi/3))-Rs*u(5)-p*u(6)*(Ld*u(4)+phis))/Lq
  dtheta_dt : Fcn  Expr=u(6)
  dwm_dt : Fcn  Expr=(1.5*p*(phis*u(5)+(Ld-Lq)*u(4)*u(5))-u(8)-F*u(6))/J
  ia : Fcn  Expr=u(4)*cos(p*u(7))-u(5)*sin(p*u(7))
  ib : Fcn  Expr=u(4)*cos(p*u(7)-2*pi/3)-u(5)*sin(p*u(7)-2*pi/3)
  ic : Fcn  Expr=u(4)*cos(p*u(7)+2*pi/3)-u(5)*sin(p*u(7)+2*pi/3)
  id_iq_wm_theta : Integrator  InitialCondition=[0;0;0;0]
  measurement : Mux  Inputs=8
  theta_m : Fcn  Expr=u(7)
  v_state_load : Mux  Inputs=3
  vd_actual : Fcn  Expr=(2/3)*(u(1)*cos(p*u(7))+u(2)*cos(p*u(7)-2*pi/3)+u(3)*cos(p*u(7)+2*pi/3))
  vq_actual : Fcn  Expr=(-2/3)*(u(1)*sin(p*u(7))+u(2)*sin(p*u(7)-2*pi/3)+u(3)*sin(p*u(7)+2*pi/3))
  wm : Fcn  Expr=u(6)
  电压观测 : Mux  Inputs=2
  电流占位电压 : Constant  Value=[0 0 0]
  电流占位转矩 : Constant  Value=0
  电流状态 : Mux  Inputs=3
  记录_obs_state : ToWorkspace  VariableName=obs_state  SaveFormat=Timeseries  SampleTime=timing_control_sample
  记录_obs_torque_fast : ToWorkspace  VariableName=obs_torque_fast  SaveFormat=Timeseries  SampleTime=T
  记录_obs_vdq_fast : ToWorkspace  VariableName=obs_vdq_fast  SaveFormat=Timeseries  SampleTime=T
  measurement_vector : Outport
  Iabc : Outport  Port=2
  tag scope: DeadMotorState=global
  wires:
  Vabc/1 -> v_state_load/1
  id_iq_wm_theta/1 -> v_state_load/2, 记录_obs_state/1, 电流状态/2, [DeadMotorState]
  load_torque/1 -> v_state_load/3
  v_state_load/1 -> did_dt/1, diq_dt/1, dwm_dt/1, dtheta_dt/1, wm/1, theta_m/1, Te/1, vq_actual/1, vd_actual/1
  did_dt/1 -> derivatives/1
  diq_dt/1 -> derivatives/2
  dwm_dt/1 -> derivatives/3
  dtheta_dt/1 -> derivatives/4
  derivatives/1 -> id_iq_wm_theta/1
  ia/1 -> measurement/1, current_vector/1
  ib/1 -> measurement/2, current_vector/2
  ic/1 -> measurement/3, current_vector/3
  wm/1 -> measurement/4
  theta_m/1 -> measurement/5
  Te/1 -> measurement/6, 记录_obs_torque_fast/1
  vq_actual/1 -> measurement/7, 电压观测/2
  vd_actual/1 -> measurement/8, 电压观测/1
  measurement/1 -> measurement_vector/1
  current_vector/1 -> Iabc/1
  电压观测/1 -> 记录_obs_vdq_fast/1
  电流占位电压/1 -> 电流状态/1
  电流占位转矩/1 -> 电流状态/3
  电流状态/1 -> ia/1, ib/1, ic/1

== system PMSM_SMO_ClosedLoop/Subsystem ==
  theta_m : Inport
  Constant : Constant  Value=2*pi
  Gain1 : Gain  Gain=p
  Mod : Math  Operator=mod
  Scope : Scope
      settings: DataLoggingVariableName=ScopeData12
  theta_e : Outport
  wires:
  Constant/1 -> Mod/2
  Mod/1 -> theta_e/1
  Gain1/1 -> Mod/1
  theta_m/1 -> Scope/1, Gain1/1

== system PMSM_SMO_ClosedLoop/Three-Phase V-I Measurement ==
  Vabc : Inport
  Iabc : Inport  Port=2
  Vab : Fcn  Expr=u(1)-u(2)
  Vbc : Fcn  Expr=u(2)-u(3)
  Vca : Fcn  Expr=u(3)-u(1)
  line_voltage : Mux  Inputs=3
  Vab_Vbc_Vca : Outport
  Iabc_measured : Outport  Port=2
  Vabc_to_motor : Outport  Port=3
  wires:
  Vabc/1 -> Vab/1, Vbc/1, Vca/1, Vabc_to_motor/1
  Vab/1 -> line_voltage/1
  Vbc/1 -> line_voltage/2
  Vca/1 -> line_voltage/3
  line_voltage/1 -> Vab_Vbc_Vca/1
  Iabc/1 -> Iabc_measured/1

== system PMSM_SMO_ClosedLoop/Universal Bridge ==
  note: Ideal switching bridge: [AH AL BH BL CH CL]. Complementary gates only.
      | Floating star neutral; no device losses, dead time or DC-link dynamics.
  six_gates : Inport
  Vdc : Inport  Port=2
  double gates : DataTypeConversion  OutDataTypeStr=double  SaturateOnIntegerOverflow=off  RndMeth=Floor
  gates_and_bus : Mux  Inputs=2
  phase_A : Fcn  Expr=u(7)*(2*(u(1)-u(2))-(u(3)-u(4))-(u(5)-u(6)))/6
  phase_B : Fcn  Expr=u(7)*(2*(u(3)-u(4))-(u(1)-u(2))-(u(5)-u(6)))/6
  phase_C : Fcn  Expr=u(7)*(2*(u(5)-u(6))-(u(1)-u(2))-(u(3)-u(4)))/6
  phase_voltage : Mux  Inputs=3
  事件时钟 : DigitalClock  SampleTime=dead_h
  桥选择 : VariantSource  VariantControls={dead_gate_on==1, dead_gate_on==0}
  相电压向量 : Reshape
  空白保留 : Terminator
  续流 : MATLAB Function  TreatAsAtomicUnit=on
  续流参数 : Constant  Value=dead_bridge_cfg
  记录_obs_dead_bridge : ToWorkspace  VariableName=obs_dead_bridge  SaveFormat=Timeseries  SampleTime=T
  记录_obs_dead_gates : ToWorkspace  VariableName=obs_dead_gates  SaveFormat=Timeseries  SampleTime=dead_h
      settings: MaxDataPoints=4000
  记录_obs_dead_requested : ToWorkspace  VariableName=obs_dead_requested  SaveFormat=Timeseries  SampleTime=dead_h
      settings: MaxDataPoints=4000
  门极参数 : Constant  Value=dead_gate_cfg
  门极向量 : Reshape
  门极死区 : MATLAB Function  TreatAsAtomicUnit=on
  门极选择 : VariantSource  VariantControls={dead_gate_on==1, dead_gate_on==0}
  Vabc : Outport
  tag scope: ObsFreewheel=global, SWact=global
  wires:
  six_gates/1 -> double gates/1
  double gates/1 -> gates_and_bus/1, 门极死区/2(request), 记录_obs_dead_requested/1, 门极选择/2
  Vdc/1 -> gates_and_bus/2, 续流/3(Vdc)
  gates_and_bus/1 -> phase_A/1, phase_B/1, phase_C/1
  phase_A/1 -> phase_voltage/1
  phase_B/1 -> phase_voltage/2
  phase_C/1 -> phase_voltage/3
  phase_voltage/1 -> 桥选择/2
  事件时钟/1 -> 门极死区/1(t)
  门极参数/1 -> 门极死区/3(cfg)
  门极死区/2(blank) -> 空白保留/1
  门极死区/1(gates) -> 门极向量/1
  门极向量/1 -> 门极选择/1
  门极选择/1 -> [SWact], 记录_obs_dead_gates/1, 续流/1(gates)
  [DeadMotorState] -> 续流/2(state)
  续流参数/1 -> 续流/4(cfg)
  续流/1(phase) -> 相电压向量/1
  相电压向量/1 -> 桥选择/1
  桥选择/1 -> Vabc/1
  续流/2(diagnostic) -> [ObsFreewheel], 记录_obs_dead_bridge/1

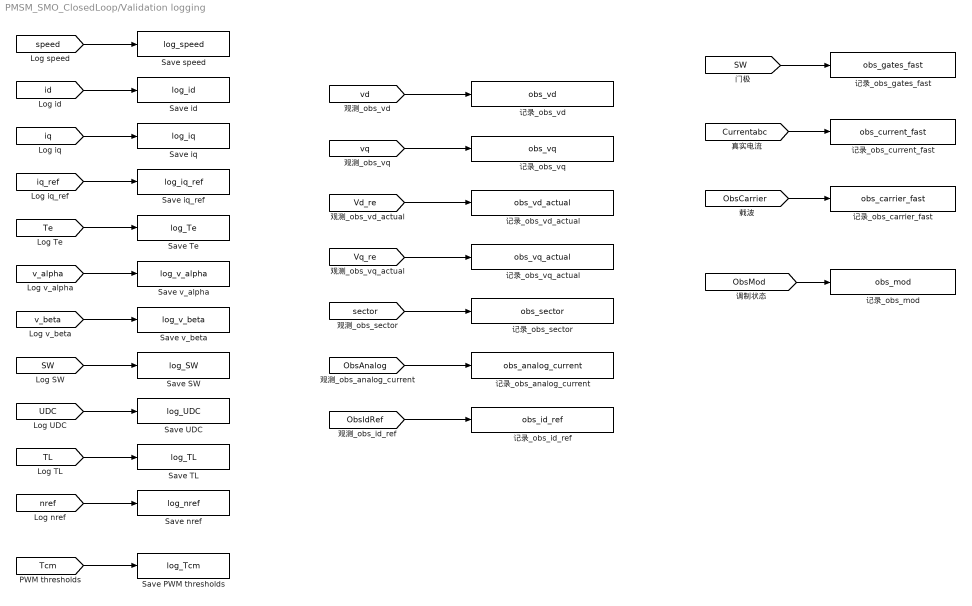
== system PMSM_SMO_ClosedLoop/Validation logging ==
  Save PWM thresholds : ToWorkspace  VariableName=log_Tcm  SaveFormat=Timeseries  SampleTime=timing_control_sample
  Save SW : ToWorkspace  VariableName=log_SW  SaveFormat=Timeseries  SampleTime=timing_control_sample
  Save TL : ToWorkspace  VariableName=log_TL  SaveFormat=Timeseries  SampleTime=timing_control_sample
  Save Te : ToWorkspace  VariableName=log_Te  SaveFormat=Timeseries  SampleTime=timing_control_sample
  Save UDC : ToWorkspace  VariableName=log_UDC  SaveFormat=Timeseries  SampleTime=timing_control_sample
  Save id : ToWorkspace  VariableName=log_id  SaveFormat=Timeseries  SampleTime=timing_control_sample
  Save iq : ToWorkspace  VariableName=log_iq  SaveFormat=Timeseries  SampleTime=timing_control_sample
  Save iq_ref : ToWorkspace  VariableName=log_iq_ref  SaveFormat=Timeseries  SampleTime=timing_control_sample
  Save nref : ToWorkspace  VariableName=log_nref  SaveFormat=Timeseries  SampleTime=timing_control_sample
  Save speed : ToWorkspace  VariableName=log_speed  SaveFormat=Timeseries  SampleTime=timing_control_sample
  Save v_alpha : ToWorkspace  VariableName=log_v_alpha  SaveFormat=Timeseries  SampleTime=timing_control_sample
  Save v_beta : ToWorkspace  VariableName=log_v_beta  SaveFormat=Timeseries  SampleTime=timing_control_sample
  记录_obs_analog_current : ToWorkspace  VariableName=obs_analog_current  SaveFormat=Timeseries  SampleTime=timing_control_sample
  记录_obs_carrier_fast : ToWorkspace  VariableName=obs_carrier_fast  SaveFormat=Timeseries  SampleTime=T
  记录_obs_current_fast : ToWorkspace  VariableName=obs_current_fast  SaveFormat=Timeseries  SampleTime=T
  记录_obs_gates_fast : ToWorkspace  VariableName=obs_gates_fast  SaveFormat=Timeseries  SampleTime=T
  记录_obs_id_ref : ToWorkspace  VariableName=obs_id_ref  SaveFormat=Timeseries  SampleTime=timing_control_sample
  记录_obs_mod : ToWorkspace  VariableName=obs_mod  SaveFormat=Timeseries  SampleTime=timing_control_sample
  记录_obs_sector : ToWorkspace  VariableName=obs_sector  SaveFormat=Timeseries  SampleTime=timing_control_sample
  记录_obs_vd : ToWorkspace  VariableName=obs_vd  SaveFormat=Timeseries  SampleTime=timing_control_sample
  记录_obs_vd_actual : ToWorkspace  VariableName=obs_vd_actual  SaveFormat=Timeseries  SampleTime=timing_control_sample
  记录_obs_vq : ToWorkspace  VariableName=obs_vq  SaveFormat=Timeseries  SampleTime=timing_control_sample
  记录_obs_vq_actual : ToWorkspace  VariableName=obs_vq_actual  SaveFormat=Timeseries  SampleTime=timing_control_sample
  wires:
  [speed] -> Save speed/1
  [id] -> Save id/1
  [iq] -> Save iq/1
  [iq_ref] -> Save iq_ref/1
  [Te] -> Save Te/1
  [v_alpha] -> Save v_alpha/1
  [v_beta] -> Save v_beta/1
  [SW] -> Save SW/1
  [UDC] -> Save UDC/1
  [TL] -> Save TL/1
  [nref] -> Save nref/1
  [Tcm] -> Save PWM thresholds/1
  [vd] -> 记录_obs_vd/1
  [vq] -> 记录_obs_vq/1
  [Vd_re] -> 记录_obs_vd_actual/1
  [Vq_re] -> 记录_obs_vq_actual/1
  [sector] -> 记录_obs_sector/1
  [ObsAnalog] -> 记录_obs_analog_current/1
  [ObsIdRef] -> 记录_obs_id_ref/1
  [SW] -> 记录_obs_gates_fast/1
  [ObsCarrier] -> 记录_obs_carrier_fast/1
  [Currentabc] -> 记录_obs_current_fast/1
  [ObsMod] -> 记录_obs_mod/1

== system PMSM_SMO_ClosedLoop/abc to Alpha-Beta-Zero ==
  abc : Inport
  Clarke matrix : Gain  Gain=[2/3 -1/3 -1/3;0 1/sqrt(3) -1/sqrt(3);1/3 1/3 1/3]  Multiplication=Matrix(K*u)
  alpha_beta_zero : Outport
  wires:
  abc/1 -> Clarke matrix/1
  Clarke matrix/1 -> alpha_beta_zero/1

== system PMSM_SMO_ClosedLoop/dq0 to Alpha-Beta-Zero ==
  dq0 : Inport
  theta_e : Inport  Port=2
  axis_0 : Fcn  Expr=u(3)
  axis_1 : Fcn  Expr=u(1)*cos(u(4))-u(2)*sin(u(4))
  axis_2 : Fcn  Expr=u(1)*sin(u(4))+u(2)*cos(u(4))
  input_vector : Mux  Inputs=2
  result : Mux  Inputs=3
  alpha_beta_zero : Outport
  wires:
  dq0/1 -> input_vector/1
  theta_e/1 -> input_vector/2
  input_vector/1 -> axis_1/1, axis_2/1, axis_0/1
  axis_1/1 -> result/1
  axis_2/1 -> result/2
  axis_0/1 -> result/3
  result/1 -> alpha_beta_zero/1

== system PMSM_SMO_ClosedLoop/功率压降 ==
  理想 : Inport
  扣除 : Sum  Inputs=+-  SampleTime=0
  旁路 : Switch  Criteria=u2 ~= 0  SampleTime=0  SaturateOnIntegerOverflow=off  InputSameDT=off
  记录_obs_phase_actual : ToWorkspace  VariableName=obs_phase_actual  SaveFormat=Timeseries  SampleTime=T
  记录_obs_phase_ideal : ToWorkspace  VariableName=obs_phase_ideal  SaveFormat=Timeseries  SampleTime=T
  实际 : Outport
  tag scope: ObsPhaseActual=global, ObsPhaseIdeal=global
  wires:
  理想/1 -> 扣除/1, 旁路/3, [ObsPhaseIdeal], 记录_obs_phase_ideal/1
  [ObsPowerDrop] -> 扣除/2
  扣除/1 -> 旁路/1
  [ObsPowerOn] -> 旁路/2
  旁路/1 -> 实际/1, [ObsPhaseActual], 记录_obs_phase_actual/1

== system PMSM_SMO_ClosedLoop/功率观测 ==
  note: 01 理想相电压 [V]
  note: 02 实际相电压 [V]
  note: 03 平均压降 [V]
  实际相电压 : Scope
      settings: SampleTime=T  Title=实际相电压 [V]
  平均压降 : Scope
      settings: SampleTime=dt  Title=平均压降 [V]
  总览 : Scope  NumInputPorts=8
      settings: SampleTime=T  TimeSpan=0.12  ActiveDisplayString=8  Title=dq补偿 [V]
  极性保留 : Terminator
  理想相电压 : Scope
      settings: SampleTime=T  Title=理想相电压 [V]
  真实电流保留 : Terminator
  续流分组 : Demux  Outputs=[3 3 3]
  补偿分组 : Demux  Outputs=[3 2 3]
  wires:
  [ObsPhaseIdeal] -> 理想相电压/1, 总览/1
  [ObsPhaseActual] -> 实际相电压/1, 总览/2
  [ObsPowerDrop] -> 平均压降/1, 总览/3
  [ObsFreewheel] -> 续流分组/1
  续流分组/3 -> 真实电流保留/1
  [ObsDeadComp] -> 补偿分组/1
  补偿分组/3 -> 极性保留/1
  [SWact] -> 总览/4
  续流分组/1 -> 总览/5
  续流分组/2 -> 总览/6
  补偿分组/1 -> 总览/7
  补偿分组/2 -> 总览/8

== system PMSM_SMO_ClosedLoop/功率设置 ==
  三相压降 : Mux  Inputs=3
  压降1 : Fcn  Expr=dead_on*dead_us*1e-6/Ts*(u(4)+drop_on*vf)*u(1)/(abs(u(1))+blend_A)+drop_on*ron*u(1)
  压降2 : Fcn  Expr=dead_on*dead_us*1e-6/Ts*(u(4)+drop_on*vf)*u(2)/(abs(u(2))+blend_A)+drop_on*ron*u(2)
  压降3 : Fcn  Expr=dead_on*dead_us*1e-6/Ts*(u(4)+drop_on*vf)*u(3)/(abs(u(3))+blend_A)+drop_on*ron*u(3)
  去共模 : Gain  Gain=eye(3)-ones(3)/3  Multiplication=Matrix(K*u)
  启用 : Constant  Value=(~dead_gate_on)&&(dead_on||drop_on)
  周期电流 : ZeroOrderHold  SampleTime=Ts
  记录_obs_power_drop : ToWorkspace  VariableName=obs_power_drop  SaveFormat=Timeseries  SampleTime=timing_control_sample
  输入 : Mux  Inputs=2
  tag scope: ObsPowerDrop=global, ObsPowerOn=global
  wires:
  [Currentabc] -> 周期电流/1
  周期电流/1 -> 输入/1
  [UDC] -> 输入/2
  输入/1 -> 压降1/1, 压降2/1, 压降3/1
  压降1/1 -> 三相压降/1
  压降2/1 -> 三相压降/2
  压降3/1 -> 三相压降/3
  三相压降/1 -> 去共模/1
  去共模/1 -> [ObsPowerDrop], 记录_obs_power_drop/1
  启用/1 -> [ObsPowerOn]
